simulink model "model_Lab3_parta"  (R2024a)
settings: Solver=VariableStepAuto  StartTime=0.0  StopTime=90  RelTol=1e-3
values from neighbouring files (symbols this model uses):
  f0i = pdesi(2) - a1    [evalutate_controller_part_a.m]
  f0o = 2.5    [evalutate_controller_part_a.m]
  f1i = 1    [evalutate_controller_part_a.m]
  f1o = 1    [evalutate_controller_part_a.m]
  g0i = pdesi(4)/b0    [evalutate_controller_part_a.m]
  g0o = -2.45    [evalutate_controller_part_a.m]
  g1i = (pdesi(3) - a1*f0i)/b0    [evalutate_controller_part_a.m]
  g1o = -7    [evalutate_controller_part_a.m]
  k1 = -1.9731    [evalutate_controller_part_a.m]
  k2 = 0.0609    [evalutate_controller_part_a.m]
  k3 = -4.838    [evalutate_controller_part_a.m]
  tau = 0.02387    [evalutate_controller_part_a.m]
settings Model: Creator=michael  LastModifiedBy=michael

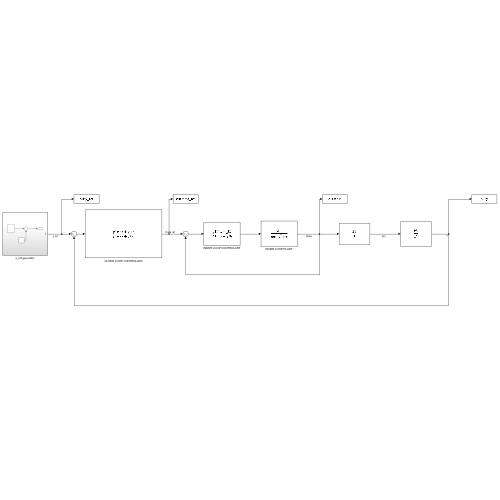
[thumbnail: Simulink's stored preview of the top-level diagram]
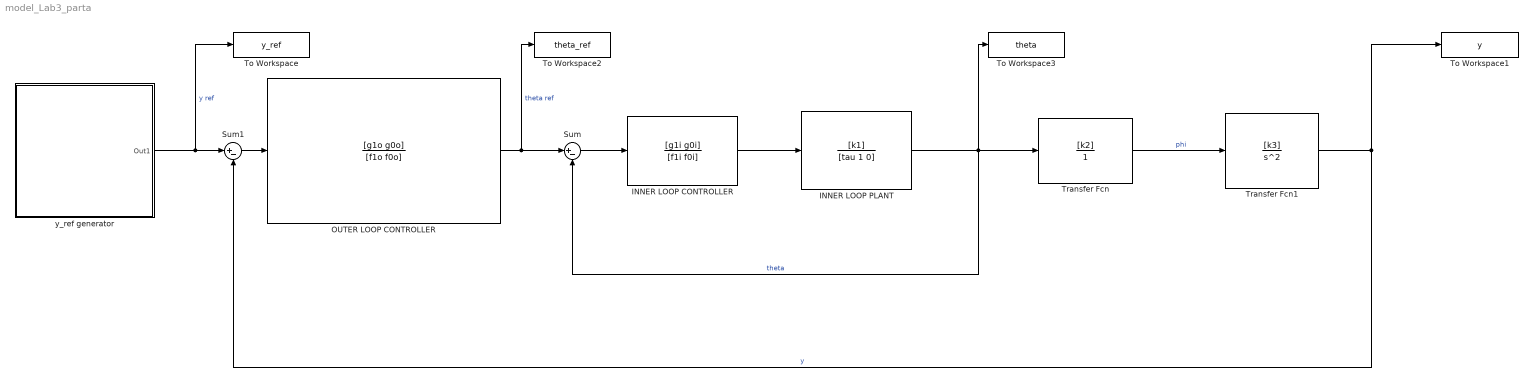
== system model_Lab3_parta ==
  INNER LOOP CONTROLLER : TransferFcn  Numerator=[g1i g0i]  Denominator=[f1i f0i]
  INNER LOOP PLANT : TransferFcn  Numerator=[k1]  Denominator=[tau 1 0]
  OUTER LOOP CONTROLLER : TransferFcn  Numerator=[g1o g0o]  Denominator=[f1o f0o]
  Sum : Sum  Inputs=|+-
  Sum1 : Sum  Inputs=|+-
  To Workspace : ToWorkspace  VariableName=y_ref  SaveFormat=Timeseries  SampleTime=-1
  To Workspace1 : ToWorkspace  VariableName=y  SaveFormat=Timeseries  SampleTime=-1
  To Workspace2 : ToWorkspace  VariableName=theta_ref  SaveFormat=Timeseries  SampleTime=-1
  To Workspace3 : ToWorkspace  VariableName=theta  SaveFormat=Timeseries  SampleTime=-1
  Transfer Fcn : TransferFcn  Numerator=[k2]  Denominator=[1]
  Transfer Fcn1 : TransferFcn  Numerator=[k3]  Denominator=[1 0 0]
  y_ref generator : Subsystem
  wires:
  INNER LOOP PLANT/1 -> Sum/2, To Workspace3/1, Transfer Fcn/1  "theta"
  INNER LOOP CONTROLLER/1 -> INNER LOOP PLANT/1
  OUTER LOOP CONTROLLER/1 -> Sum/1, To Workspace2/1  "theta ref"
  Sum/1 -> INNER LOOP CONTROLLER/1
  Transfer Fcn/1 -> Transfer Fcn1/1  "phi"
  y_ref generator/1(Out1) -> To Workspace/1, Sum1/1  "y ref"
  Sum1/1 -> OUTER LOOP CONTROLLER/1
  Transfer Fcn1/1 -> Sum1/2, To Workspace1/1  "y"

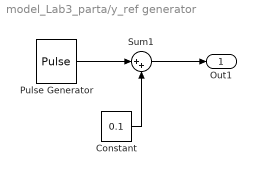
== system model_Lab3_parta/y_ref generator ==
  Constant : Constant  Value=0.1
  Pulse Generator : DiscretePulseGenerator  PulseType=Time based  Amplitude=0.15  Period=30  PulseWidth=50
  Sum1 : Sum  Inputs=|++
  Out1 : Outport
  wires:
  Constant/1 -> Sum1/2
  Pulse Generator/1 -> Sum1/1
  Sum1/1 -> Out1/1
